simulink model "ex_02_sim"  (R2024b)
settings: Solver=VariableStepAuto  StartTime=0.0  StopTime=10.0  RelTol=1e-3
values from neighbouring files (symbols this model uses):
  A = d.A    [ex_02_main.m]
  B = d.B    [ex_02_main.m]
  C = d.C    [ex_02_main.m]
  D = d.D    [ex_02_main.m]
  K = d.K    [ex_02_main.m]
undefined symbols (not defined in the file or in its folder): H, v1_gain, v1_start, v2_gain, v2_start
settings Model: Creator=54238  LastModifiedBy=54238

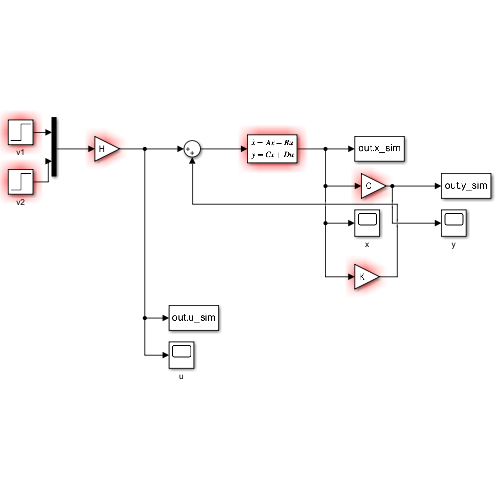
[thumbnail: Simulink's stored preview of the top-level diagram]
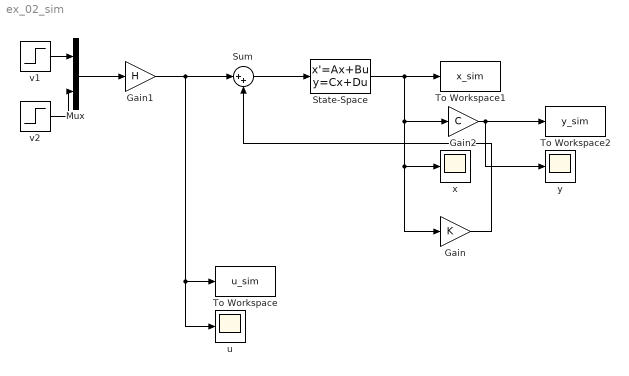
== system ex_02_sim ==
  Gain : Gain  Gain=K
  Gain1 : Gain  Gain=H
  Gain2 : Gain  Gain=C
  Mux : Mux  Inputs=2
  State-Space : StateSpace  A=A  B=B  C=C  D=D  InitialCondition=0
  Sum : Sum  Inputs=|++
  To Workspace : ToWorkspace  VariableName=u_sim  SaveFormat=Timeseries  SampleTime=-1
  To Workspace1 : ToWorkspace  VariableName=x_sim  SaveFormat=Timeseries  SampleTime=-1
  To Workspace2 : ToWorkspace  VariableName=y_sim  SaveFormat=Timeseries  SampleTime=-1
  u : Scope
  v1 : Step  Time=v1_start  After=v1_gain  SampleTime=0
  v2 : Step  Time=v2_start  After=v2_gain  SampleTime=0
  x : Scope
  y : Scope
  wires:
  v1/1 -> Mux/1
  v2/1 -> Mux/2
  Mux/1 -> Gain1/1
  Gain1/1 -> u/1, To Workspace/1, Sum/1
  Gain2/1 -> To Workspace2/1, y/1
  State-Space/1 -> Gain/1, x/1, Gain2/1, To Workspace1/1
  Sum/1 -> State-Space/1
  Gain/1 -> Sum/2
